simulink model "drone_model"  (R2022a)
settings: Solver=FixedStepAuto  StartTime=0.0  StopTime=10  FixedStep=0.005  RelTol=1e-3
InitFcn:
  | InitParameters
values from neighbouring files (symbols this model uses):
  AttDyna_Ixx = 0.0211    [InitParameters.m]
  AttDyna_Iyy = 0.0219    [InitParameters.m]
  AttDyna_Izz = 0.0366    [InitParameters.m]
  ConEfficiency_drone_cM = 1.779e-07    [InitParameters.m]
  ConEfficiency_drone_cT = 1.105e-05    [InitParameters.m]
  ConEfficiency_drone_R = 0.225    [InitParameters.m]
  PosDyna_GravityAcc = 9.8    [InitParameters.m]
  PosDyna_Mass = 1.4    [InitParameters.m]
  PowerUnit_CR = 1148    [InitParameters.m]
  PowerUnit_Tm = 0.02    [InitParameters.m]
  PowerUnit_wb = -141.4    [InitParameters.m]
undefined symbols (not defined in the file or in its folder): earthRadius, Receive, Send
libraries: simulink x5, aerolibfltsims x3, aerolibanimutils x1
settings Model: Creator=ZhangZheng  LastModifiedBy=13501
settings SolverCC: AlgebraicLoopSolver=TrustRegion
settings DebuggingCC: UnconnectedInputMsg=warning  UnconnectedOutputMsg=warning  UnconnectedLineMsg=warning  SFMachineParentedDataDiag=warning  ArithmeticOperatorsInVariantConditions=warning
settings SFSimCC: SimUseLocalCustomCode=off  CustomCodeUndefinedFunction=UseInterfaceOnly
settings RTWCC: RTWUseLocalCustomCode=off

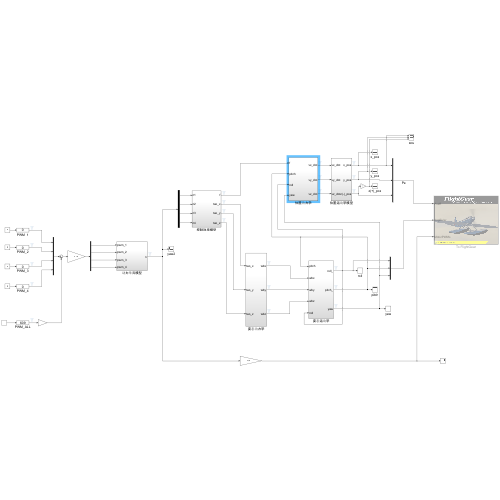
[thumbnail: Simulink's stored preview of the top-level diagram]
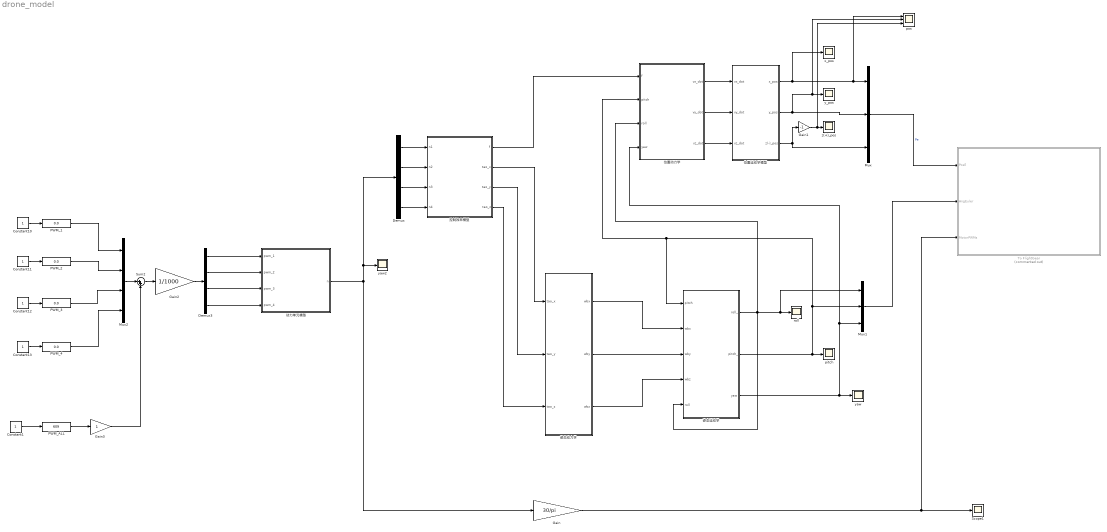
== system drone_model ==
  Constant{1,10..13} (5 alike) : Constant
  Demux : Demux
  Demux3 : Demux
  Gain : Gain  Gain=30/pi
  Gain1 : Gain  Gain=-1
  Gain2 : Gain  Gain=1/1000
  Gain3 : Gain
  Mux : Mux  Inputs=3
  Mux1 : Mux  Inputs=3
  Mux2 : Mux
  PWM_{1..4} (4 alike) : simulink/Math Operations/Slider Gain  gain=0.0  low=0  high=1000
  PWM_ALL : simulink/Math Operations/Slider Gain  gain=609  low=0  high=1000
  Scope1 : Scope
  Sum2 : Sum  Inputs=|++
  To FlightGear : Subsystem  Commented=on
      mask Display: image('./icon/FlightGear.png');
  pitch : Scope
  pos : Scope  NumInputPorts=3
  roll : Scope
  x_pos : Scope
  y_pos : Scope
  yaw : Scope
  yaw2 : Scope
  z(+)_pos : Scope
  位置动力学 : Subsystem
  位置运动学模型 : Subsystem
  动力单元模型 : Subsystem
  姿态动力学 : Subsystem
  姿态运动学 : Subsystem
  控制效率模型 : Subsystem
  wires:
  Demux/1 -> 控制效率模型/1(n1)
  Demux/2 -> 控制效率模型/2(n2)
  Demux/3 -> 控制效率模型/3(n3)
  Demux/4 -> 控制效率模型/4(n4)
  控制效率模型/1(f) -> 位置动力学/1(f)
  控制效率模型/2(tao_x) -> 姿态动力学/1(tao_x)
  控制效率模型/3(tao_y) -> 姿态动力学/2(tao_y)
  控制效率模型/4(tao_z) -> 姿态动力学/3(tao_z)
  姿态动力学/1(wbx) -> 姿态运动学/2(wbx)
  姿态动力学/2(wby) -> 姿态运动学/3(wby)
  姿态动力学/3(wbz) -> 姿态运动学/4(wbz)
  姿态运动学/2(pitch_) -> Mux1/2, 姿态运动学/1(pitch), 位置动力学/2(pitch), pitch/1
  姿态运动学/1(roll_) -> Mux1/1, roll/1, 姿态运动学/5(roll), 位置动力学/3(roll)
  姿态运动学/3(yaw) -> Mux1/3, 位置动力学/4(yaw), yaw/1
  Mux/1 -> To FlightGear/1(PosE)  "Pe"
  Gain/1 -> Scope1/1, To FlightGear/3(MotorPWMs)
  Mux1/1 -> To FlightGear/2(AngEuler)
  Gain1/1 -> pos/3, z(+)_pos/1
  PWM_ALL/1 -> Gain3/1
  Constant1/1 -> PWM_ALL/1
  Gain3/1 -> Sum2/2
  Constant10/1 -> PWM_1/1
  Constant11/1 -> PWM_2/1
  Constant12/1 -> PWM_3/1
  Constant13/1 -> PWM_4/1
  Mux2/1 -> Sum2/1
  Sum2/1 -> Gain2/1
  Demux3/1 -> 动力单元模型/1(pwm_1)
  Demux3/2 -> 动力单元模型/2(pwm_2)
  Demux3/3 -> 动力单元模型/3(pwm_3)
  Demux3/4 -> 动力单元模型/4(pwm_4)
  Gain2/1 -> Demux3/1
  动力单元模型/1(n) -> Gain/1, yaw2/1, Demux/1
  PWM_1/1 -> Mux2/1
  PWM_2/1 -> Mux2/2
  PWM_3/1 -> Mux2/3
  PWM_4/1 -> Mux2/4
  位置运动学模型/1(x_pos) -> pos/1, Mux/1, x_pos/1
  位置运动学模型/2(y_pos) -> Mux/2, pos/2, y_pos/1
  位置运动学模型/3(z(-)_pos) -> Mux/3, Gain1/1
  位置动力学/1(vx_dot) -> 位置运动学模型/1(vx_dot)
  位置动力学/2(vy_dot) -> 位置运动学模型/2(vy_dot)
  位置动力学/3(vz_dot) -> 位置运动学模型/3(vz_dot)

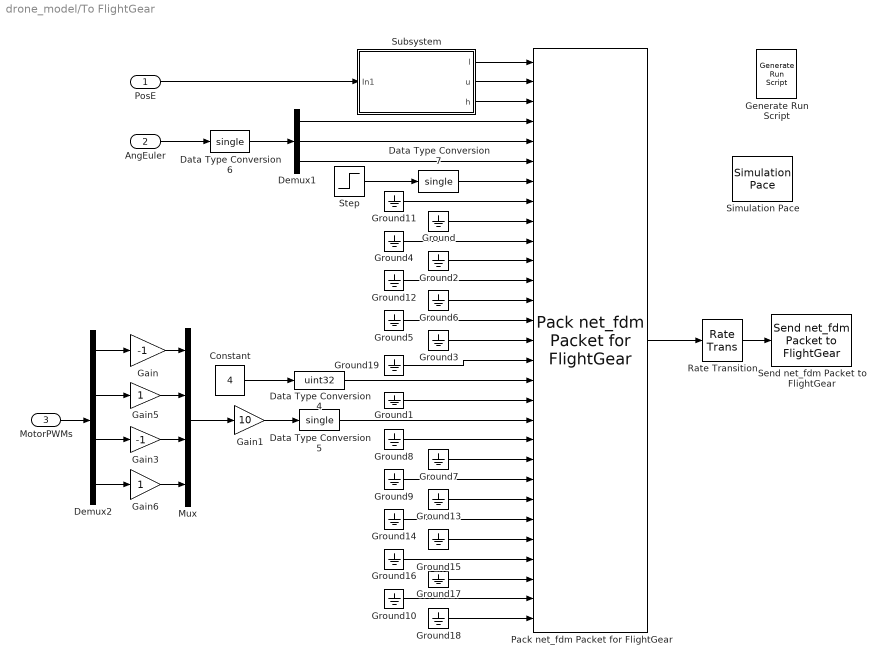
== system drone_model/To FlightGear ==
  PosE : Inport
  AngEuler : Inport  Port=2
  MotorPWMs : Inport  Port=3
  Constant : Constant  Value=4
  Data Type Conversion4 : DataTypeConversion  OutDataTypeStr=uint32  SaturateOnIntegerOverflow=off  RndMeth=Floor
  Data Type Conversion5 : DataTypeConversion  OutDataTypeStr=single  SaturateOnIntegerOverflow=off  RndMeth=Floor
  Data Type Conversion6 : DataTypeConversion  OutDataTypeStr=single  SaturateOnIntegerOverflow=off  RndMeth=Floor
  Data Type Conversion7 : DataTypeConversion  OutDataTypeStr=single  SaturateOnIntegerOverflow=off  RndMeth=Floor
  Demux1 : Demux  Outputs=3
  Demux2 : Demux
  Gain : Gain  Gain=-1
  Gain1 : Gain  Gain=10
  Gain3 : Gain  Gain=-1
  Gain5 : Gain
  Gain6 : Gain
  Generate Run Script : aerolibfltsims/Generate Run Script  OutputFileName=runfg.bat  FlightGearBaseDirectory=E:\PX4PSP\FlightGear 2016.1.2  GeometryModelName=myownUAV  DestinationPort=5502  OriginAddress=127.0.0.1  OriginPort=5505  LocalAddress=127.0.0.1  AirportId=KSFO  RunwayId=0  InitialAltitude=0  InitialHeading=0  OffsetDistance=0  OffsetAzimuth=0  GenerateFile=off  Architecture=Win64  dataFlow=Send-Receive
  Ground{,1..19} (20 alike) : Ground
  Mux : Mux
  Pack net_fdm Packet for FlightGear : aerolibfltsims/Pack net_fdm Packet for FlightGear  FlightGearVersion=v2016.1  ShowPositionAttitudeInputs=on  ShowVelocityAccelerationInputs=off  ShowControlSurfacePositionInputs=on  ShowEngineFuelInputs=on  ShowLandingGearInputs=off  ShowEnvironmentInputs=off  SampleTime=0.01
      settings: SourceProductBaseCode=AE
  Rate Transition : RateTransition
  Send net_fdm Packet to FlightGear : aerolibfltsims/Send net_fdm Packet to FlightGear  DestinationIpAddress=127.0.0.1  DestinationPort=5502  LocalIpPort=-1  varLen=off  SampleTime=0.005
      settings: SourceProductBaseCode=AE
  Simulation Pace : aerolibanimutils/Simulation Pace  SimulationPace=1  SleepMode=MATLAB Thread  OutputPaceError=off  SampleTime=-1
      settings: AttributesFormatString=%<SimulationPace> sec/sec
  Step : Step  Time=5  SampleTime=0
  Subsystem : Subsystem
  wires:
  Pack net_fdm Packet for FlightGear/1 -> Rate Transition/1
  Data Type Conversion7/1 -> Pack net_fdm Packet for FlightGear/7
  Ground8/1 -> Pack net_fdm Packet for FlightGear/20
  Ground/1 -> Pack net_fdm Packet for FlightGear/9
  Ground7/1 -> Pack net_fdm Packet for FlightGear/21
  Ground9/1 -> Pack net_fdm Packet for FlightGear/22
  Ground13/1 -> Pack net_fdm Packet for FlightGear/23
  Ground14/1 -> Pack net_fdm Packet for FlightGear/24
  Ground15/1 -> Pack net_fdm Packet for FlightGear/25
  Ground16/1 -> Pack net_fdm Packet for FlightGear/26
  Ground17/1 -> Pack net_fdm Packet for FlightGear/27
  Ground10/1 -> Pack net_fdm Packet for FlightGear/28
  Ground18/1 -> Pack net_fdm Packet for FlightGear/29
  Step/1 -> Data Type Conversion7/1
  Data Type Conversion4/1 -> Pack net_fdm Packet for FlightGear/17
  Ground1/1 -> Pack net_fdm Packet for FlightGear/18
  Ground3/1 -> Pack net_fdm Packet for FlightGear/15
  Ground5/1 -> Pack net_fdm Packet for FlightGear/14
  Ground6/1 -> Pack net_fdm Packet for FlightGear/13
  Ground4/1 -> Pack net_fdm Packet for FlightGear/10
  Ground11/1 -> Pack net_fdm Packet for FlightGear/8
  Constant/1 -> Data Type Conversion4/1
  Data Type Conversion5/1 -> Pack net_fdm Packet for FlightGear/19
  Ground2/1 -> Pack net_fdm Packet for FlightGear/11
  Ground12/1 -> Pack net_fdm Packet for FlightGear/12
  AngEuler/1 -> Data Type Conversion6/1
  MotorPWMs/1 -> Demux2/1
  Mux/1 -> Gain1/1
  Demux2/1 -> Gain/1
  Demux2/3 -> Gain3/1
  Gain/1 -> Mux/1
  Gain3/1 -> Mux/3
  Demux2/2 -> Gain5/1
  Gain5/1 -> Mux/2
  Demux2/4 -> Gain6/1
  Gain6/1 -> Mux/4
  Rate Transition/1 -> Send net_fdm Packet to FlightGear/1
  PosE/1 -> Subsystem/1(In1)
  Subsystem/1("l ") -> Pack net_fdm Packet for FlightGear/1
  Subsystem/2(u) -> Pack net_fdm Packet for FlightGear/2
  Subsystem/3(h) -> Pack net_fdm Packet for FlightGear/3
  Ground19/1 -> Pack net_fdm Packet for FlightGear/16
  Demux1/1 -> Pack net_fdm Packet for FlightGear/4
  Demux1/2 -> Pack net_fdm Packet for FlightGear/5
  Demux1/3 -> Pack net_fdm Packet for FlightGear/6
  Data Type Conversion6/1 -> Demux1/1
  Gain1/1 -> Data Type Conversion5/1

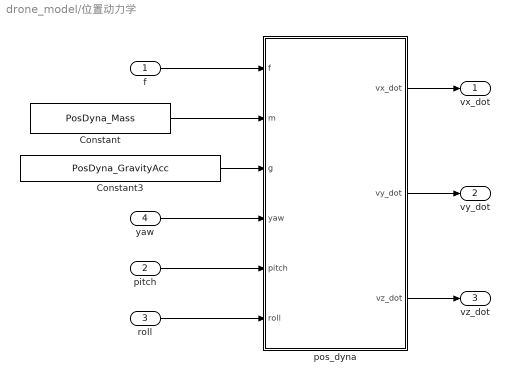
== system drone_model/位置动力学 ==
  f : Inport
  pitch : Inport  Port=2
  roll : Inport  Port=3
  yaw : Inport  Port=4
  Constant : Constant  Value=PosDyna_Mass
  Constant3 : Constant  Value=PosDyna_GravityAcc
  pos_dyna : MATLAB Function  TreatAsAtomicUnit=on
  vx_dot : Outport  VectorParamsAs1DForOutWhenUnconnected=off
  vy_dot : Outport  Port=2  VectorParamsAs1DForOutWhenUnconnected=off
  vz_dot : Outport  Port=3  VectorParamsAs1DForOutWhenUnconnected=off
  wires:
  pos_dyna/1(vx_dot) -> vx_dot/1
  Constant/1 -> pos_dyna/2(m)
  pos_dyna/3(vz_dot) -> vz_dot/1
  pos_dyna/2(vy_dot) -> vy_dot/1
  Constant3/1 -> pos_dyna/3(g)
  yaw/1 -> pos_dyna/4(yaw)
  pitch/1 -> pos_dyna/5(pitch)
  roll/1 -> pos_dyna/6(roll)
  f/1 -> pos_dyna/1(f)

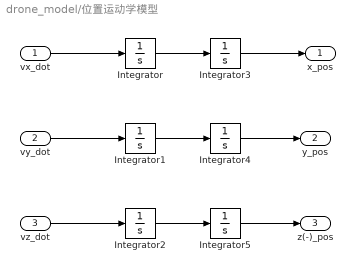
== system drone_model/位置运动学模型 ==
  vx_dot : Inport
  vy_dot : Inport  Port=2
  vz_dot : Inport  Port=3
  Integrator{,1..5} (6 alike) : Integrator
  x_pos : Outport  VectorParamsAs1DForOutWhenUnconnected=off
  y_pos : Outport  Port=2  VectorParamsAs1DForOutWhenUnconnected=off
  z(-)_pos : Outport  Port=3  VectorParamsAs1DForOutWhenUnconnected=off
  wires:
  Integrator1/1 -> Integrator4/1
  Integrator/1 -> Integrator3/1
  Integrator2/1 -> Integrator5/1
  vz_dot/1 -> Integrator2/1
  Integrator5/1 -> z(-)_pos/1
  vx_dot/1 -> Integrator/1
  vy_dot/1 -> Integrator1/1
  Integrator4/1 -> y_pos/1
  Integrator3/1 -> x_pos/1

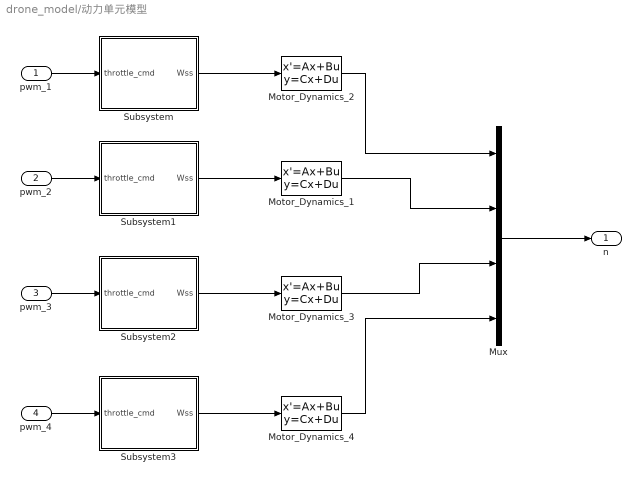
== system drone_model/动力单元模型 ==
  pwm_1 : Inport
  pwm_2 : Inport  Port=2
  pwm_3 : Inport  Port=3
  pwm_4 : Inport  Port=4
  Motor_Dynamics_{1..4} (4 alike) : StateSpace  A=-1/PowerUnit_Tm  C=1/PowerUnit_Tm  D=0  InitialCondition=557.142*PowerUnit_Tm
  Mux : Mux
  Subsystem : Subsystem
  Subsystem1 : Subsystem
  Subsystem2 : Subsystem
  Subsystem3 : Subsystem
  n : Outport  VectorParamsAs1DForOutWhenUnconnected=off
  wires:
  pwm_4/1 -> Subsystem3/1("throttle_cmd ")
  pwm_2/1 -> Subsystem1/1("throttle_cmd ")
  Subsystem2/1(Wss) -> Motor_Dynamics_3/1
  Mux/1 -> n/1
  Subsystem1/1(Wss) -> Motor_Dynamics_1/1
  pwm_3/1 -> Subsystem2/1("throttle_cmd ")
  Motor_Dynamics_4/1 -> Mux/4
  Subsystem3/1(Wss) -> Motor_Dynamics_4/1
  Motor_Dynamics_2/1 -> Mux/1
  pwm_1/1 -> Subsystem/1("throttle_cmd ")
  Motor_Dynamics_3/1 -> Mux/3
  Subsystem/1(Wss) -> Motor_Dynamics_2/1
  Motor_Dynamics_1/1 -> Mux/2

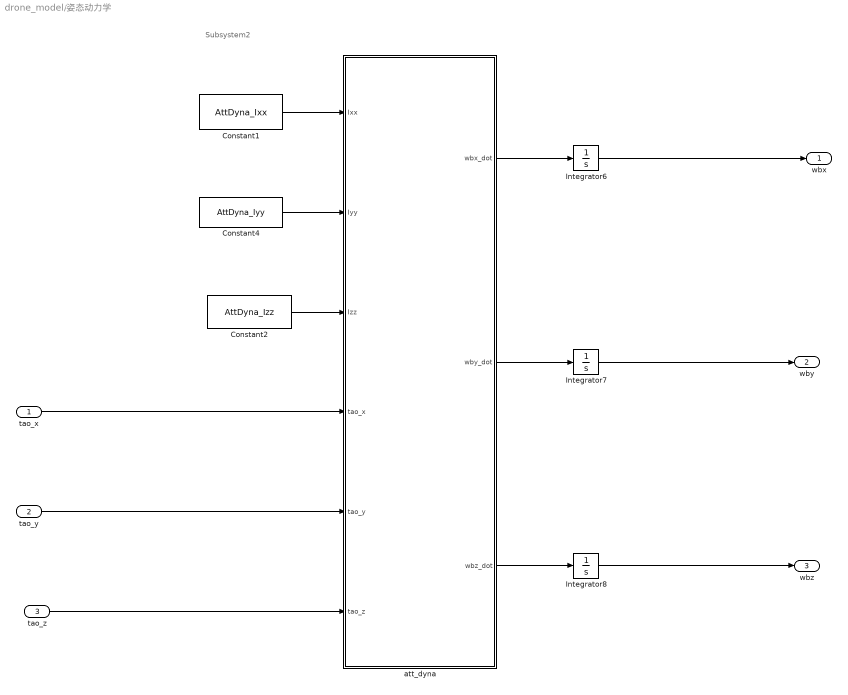
== system drone_model/姿态动力学 ==
  note: Subsystem2
  tao_x : Inport
  tao_y : Inport  Port=2
  tao_z : Inport  Port=3
  Constant1 : Constant  Value=AttDyna_Ixx
  Constant2 : Constant  Value=AttDyna_Izz
  Constant4 : Constant  Value=AttDyna_Iyy
  Integrator6 : Integrator
  Integrator7 : Integrator
  Integrator8 : Integrator
  att_dyna : MATLAB Function  TreatAsAtomicUnit=on
  wbx : Outport  VectorParamsAs1DForOutWhenUnconnected=off
  wby : Outport  Port=2  VectorParamsAs1DForOutWhenUnconnected=off
  wbz : Outport  Port=3  VectorParamsAs1DForOutWhenUnconnected=off
  wires:
  att_dyna/3(wbz_dot) -> Integrator8/1
  att_dyna/2(wby_dot) -> Integrator7/1
  att_dyna/1(wbx_dot) -> Integrator6/1
  tao_y/1 -> att_dyna/5(tao_y)
  tao_z/1 -> att_dyna/6(tao_z)
  tao_x/1 -> att_dyna/4(tao_x)
  Integrator8/1 -> wbz/1
  Integrator6/1 -> wbx/1
  Integrator7/1 -> wby/1
  Constant2/1 -> att_dyna/3(Izz)
  Constant4/1 -> att_dyna/2(Iyy)
  Constant1/1 -> att_dyna/1(Ixx)

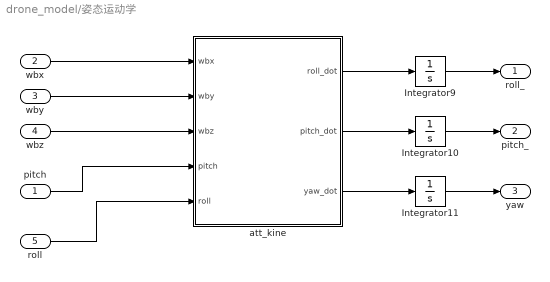
== system drone_model/姿态运动学 ==
  pitch : Inport
  wbx : Inport  Port=2
  wby : Inport  Port=3
  wbz : Inport  Port=4
  roll : Inport  Port=5
  Integrator10 : Integrator
  Integrator11 : Integrator
  Integrator9 : Integrator
  att_kine : MATLAB Function  TreatAsAtomicUnit=on
  roll_ : Outport  VectorParamsAs1DForOutWhenUnconnected=off
  pitch_ : Outport  Port=2  VectorParamsAs1DForOutWhenUnconnected=off
  yaw : Outport  Port=3  VectorParamsAs1DForOutWhenUnconnected=off
  wires:
  Integrator9/1 -> roll_/1
  att_kine/1(roll_dot) -> Integrator9/1
  att_kine/2(pitch_dot) -> Integrator10/1
  Integrator11/1 -> yaw/1
  Integrator10/1 -> pitch_/1
  att_kine/3(yaw_dot) -> Integrator11/1
  roll/1 -> att_kine/5(roll)
  pitch/1 -> att_kine/4(pitch)
  wbx/1 -> att_kine/1(wbx)
  wby/1 -> att_kine/2(wby)
  wbz/1 -> att_kine/3(wbz)

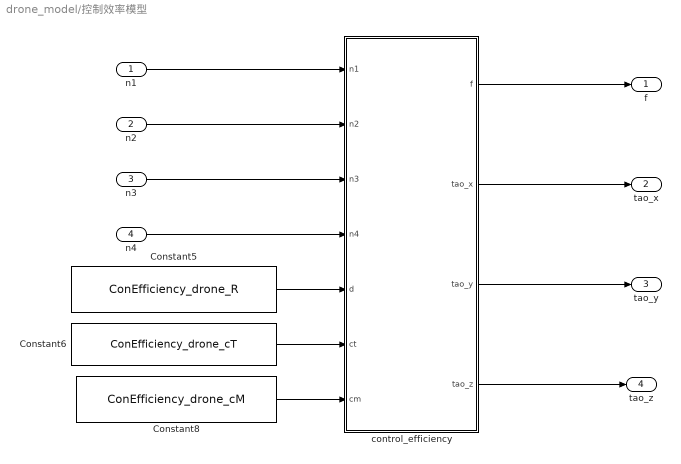
== system drone_model/控制效率模型 ==
  n1 : Inport
  n2 : Inport  Port=2
  n3 : Inport  Port=3
  n4 : Inport  Port=4
  Constant5 : Constant  Value=ConEfficiency_drone_R
  Constant6 : Constant  Value=ConEfficiency_drone_cT
  Constant8 : Constant  Value=ConEfficiency_drone_cM
  control_efficiency : MATLAB Function  TreatAsAtomicUnit=on
  f : Outport  VectorParamsAs1DForOutWhenUnconnected=off
  tao_x : Outport  Port=2  VectorParamsAs1DForOutWhenUnconnected=off
  tao_y : Outport  Port=3  VectorParamsAs1DForOutWhenUnconnected=off
  tao_z : Outport  Port=4  VectorParamsAs1DForOutWhenUnconnected=off
  wires:
  control_efficiency/1(f) -> f/1
  control_efficiency/4(tao_z) -> tao_z/1
  n4/1 -> control_efficiency/4(n4)
  control_efficiency/2(tao_x) -> tao_x/1
  n3/1 -> control_efficiency/3(n3)
  control_efficiency/3(tao_y) -> tao_y/1
  n2/1 -> control_efficiency/2(n2)
  Constant8/1 -> control_efficiency/7(cm)
  n1/1 -> control_efficiency/1(n1)
  Constant5/1 -> control_efficiency/5(d)
  Constant6/1 -> control_efficiency/6(ct)

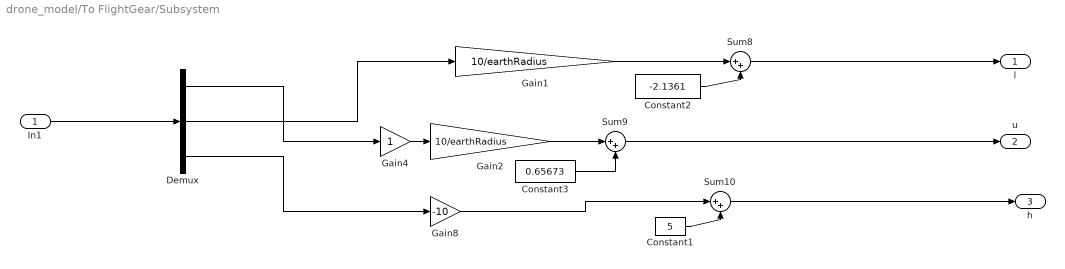
== system drone_model/To FlightGear/Subsystem ==
  In1 : Inport
  Constant1 : Constant  Value=5  VectorParams1D=off
  Constant2 : Constant  Value=-2.1361  VectorParams1D=off
  Constant3 : Constant  Value=0.65673  VectorParams1D=off
  Demux : Demux  Outputs=3
  Gain1 : Gain  Gain=10/earthRadius
  Gain2 : Gain  Gain=10/earthRadius
  Gain4 : Gain
  Gain8 : Gain  Gain=-10
  Sum10 : Sum  Inputs=|++
  Sum8 : Sum  Inputs=|++
  Sum9 : Sum  Inputs=|++
  "l " : Outport  VectorParamsAs1DForOutWhenUnconnected=off
  u : Outport  Port=2  VectorParamsAs1DForOutWhenUnconnected=off
  h : Outport  Port=3  VectorParamsAs1DForOutWhenUnconnected=off
  wires:
  Constant3/1 -> Sum9/2
  Constant1/1 -> Sum10/2
  Demux/1 -> Gain4/1
  Demux/3 -> Gain8/1
  Constant2/1 -> Sum8/2
  Gain2/1 -> Sum9/1
  Gain1/1 -> Sum8/1
  Gain8/1 -> Sum10/1
  Demux/2 -> Gain1/1
  Gain4/1 -> Gain2/1
  Sum10/1 -> h/1
  Sum9/1 -> u/1
  In1/1 -> Demux/1
  Sum8/1 -> "l "/1

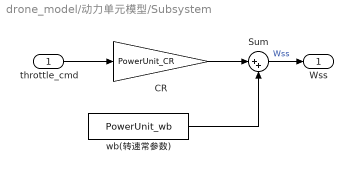
== system drone_model/动力单元模型/Subsystem ==
  "throttle_cmd " : Inport
  CR : Gain  Gain=PowerUnit_CR
  Sum : Sum  Inputs=|++
  wb(转速常参数) : Constant  Value=PowerUnit_wb
  Wss : Outport  VectorParamsAs1DForOutWhenUnconnected=off
  wires:
  "throttle_cmd "/1 -> CR/1
  CR/1 -> Sum/1
  wb(转速常参数)/1 -> Sum/2
  Sum/1 -> Wss/1  "Wss"

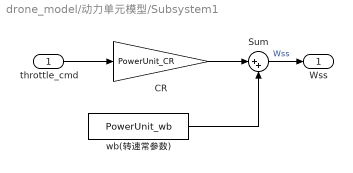
== system drone_model/动力单元模型/Subsystem1 ==
  "throttle_cmd " : Inport
  CR : Gain  Gain=PowerUnit_CR
  Sum : Sum  Inputs=|++
  wb(转速常参数) : Constant  Value=PowerUnit_wb
  Wss : Outport  VectorParamsAs1DForOutWhenUnconnected=off
  wires:
  Sum/1 -> Wss/1  "Wss"
  wb(转速常参数)/1 -> Sum/2
  CR/1 -> Sum/1
  "throttle_cmd "/1 -> CR/1

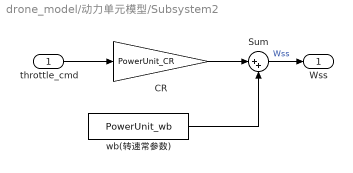
== system drone_model/动力单元模型/Subsystem2 ==
  "throttle_cmd " : Inport
  CR : Gain  Gain=PowerUnit_CR
  Sum : Sum  Inputs=|++
  wb(转速常参数) : Constant  Value=PowerUnit_wb
  Wss : Outport  VectorParamsAs1DForOutWhenUnconnected=off
  wires:
  "throttle_cmd "/1 -> CR/1
  CR/1 -> Sum/1
  wb(转速常参数)/1 -> Sum/2
  Sum/1 -> Wss/1  "Wss"

== system drone_model/动力单元模型/Subsystem3 ==
  "throttle_cmd " : Inport
  CR : Gain  Gain=PowerUnit_CR
  Sum : Sum  Inputs=|++
  wb(转速常参数) : Constant  Value=PowerUnit_wb
  Wss : Outport  VectorParamsAs1DForOutWhenUnconnected=off
  wires:
  Sum/1 -> Wss/1  "Wss"
  wb(转速常参数)/1 -> Sum/2
  CR/1 -> Sum/1
  "throttle_cmd "/1 -> CR/1

== matlab function drone_model/姿态动力学/att_dyna ==
  data: Ixx input; Iyy input; Izz input; tao_x input; tao_y input; tao_z input; wbx_dot output; wby_dot output; wbz_dot output
function [wbx_dot,wby_dot,wbz_dot] = att_dyna(Ixx,Iyy,Izz,tao_x,tao_y,tao_z)
% wb = [wbx wby wbz]';
% wb_cha = [   0 -wbz   wby;
%            wbz    0  -wbx;
%           -wby  wbx     0];
% I = [Ixx   0   0;
%        0 Iyy   0;
%        0   0 Izz];
I_inv = [1/Ixx     0     0;
             0 1/Iyy     0;
             0     0 1/Izz];
tao = [tao_x tao_y tao_z]';
% G_x = Jrp * wby * (n1+n2-n3-n4);
% G_y = Jrp * wbx * (-n1-n2+n3+n4);
% G_z = 0;  
% G = [G_x G_y G_z]';
wb_dot = I_inv * (tao);
wbx_dot = wb_dot(1,1);
wby_dot = wb_dot(2,1);
wbz_dot = wb_dot(3,1);
end

== matlab function drone_model/位置动力学/pos_dyna ==
  data: f input; vx_dot output; m input; g input; yaw input; pitch input; roll input; vy_dot output; vz_dot output
function [vx_dot,vy_dot,vz_dot] = pos_dyna(f,m,g,yaw,pitch,roll)
%位置动力学
%忽略了角速度和线速度的叉乘
%输入：拉力，重力，三个欧拉角
%输出：空间坐标系下的三个加速度
vx_dot = (sin(roll)*sin(yaw) + cos(roll)*cos(yaw)*sin(pitch))*f/m;
vy_dot = (cos(roll)*sin(pitch)*sin(yaw) - cos(yaw)*sin(roll))*f/m;
vz_dot = g-(cos(pitch)*cos(roll)*f/m);
end

== matlab function drone_model/姿态运动学/att_kine ==
  data: wbx input; roll_dot output; wby input; wbz input; pitch input; pitch_dot output; yaw_dot output; roll input
function [roll_dot,pitch_dot,yaw_dot] = att_kine(wbx,wby,wbz,pitch,roll)
%姿态运动学
%输入：机体坐标系下的三个角速度，pitch轴的角度和x轴的角度
%输出：三个欧拉角的角速率
roll_dot = wbx + tan(pitch)*sin(roll)*wby + tan(pitch)*cos(roll)*wbz;
pitch_dot = cos(roll)*wby - sin(roll)*wbz;
yaw_dot = (sin(roll)/cos(pitch))*wby + (cos(roll)/cos(pitch))*wbz;
end

== matlab function drone_model/控制效率模型/control_efficiency ==
  data: n1 input; f output; n2 input; n3 input; n4 input; tao_x output; tao_y output; tao_z output; d input; ct input; cm input
function [f,tao_x,tao_y,tao_z] = control_efficiency(n1,n2,n3,n4,d,ct,cm)
%控制效率模型
%X型机架
%3↓   1↑
%  \ /
%  / \
%2↑   4↓
%转速单位是弧度/s
f = ct*(n1^2 + n2^2 + n3^2 + n4^2);%z轴朝下，所以拉力为负
tao_x = d*ct*sin(pi/4)*(-n1^2 + n2^2 + n3^2 - n4^2) / 2;
tao_y = d*ct*sin(pi/4)*(n1^2 - n2^2 + n3^2 - n4^2) / 2;
tao_z = cm*(n1^2 + n2^2 - n3^2 - n4^2);
%十字型
% f = ct*(n1^2 + n2^2 + n3^2 + n4^2);
% tao_x = -d*ct*n2^2 + d*ct*n4^2;
% tao_y =  d*ct*n1^2 - d*ct*n3^2;
% tao_z = cm*(n1^2 - n2^2 + n3^2 - n4^2);
end
